simulink model "HW4"  (R2023b)
settings: Solver=FixedStepAuto  StartTime=0.0  StopTime=100  FixedStep=0.5  RelTol=1e-3
settings Model: Creator=ArshiaGosh  LastModifiedBy=ArshiaGosh

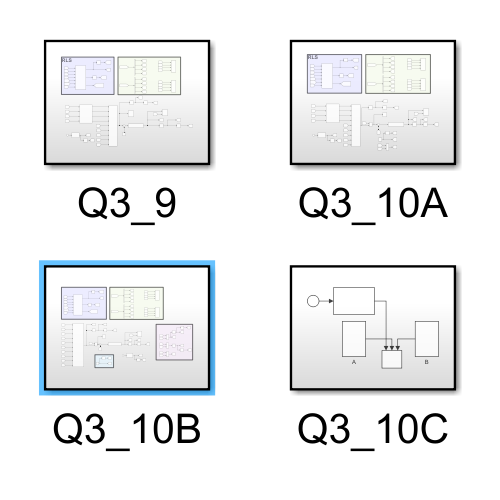
[thumbnail: Simulink's stored preview of the top-level diagram]
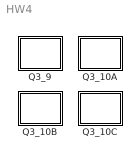
== system HW4 ==
  Q3_10A : Subsystem
  Q3_10B : Subsystem
  Q3_10C : Subsystem
  Q3_9 : Subsystem

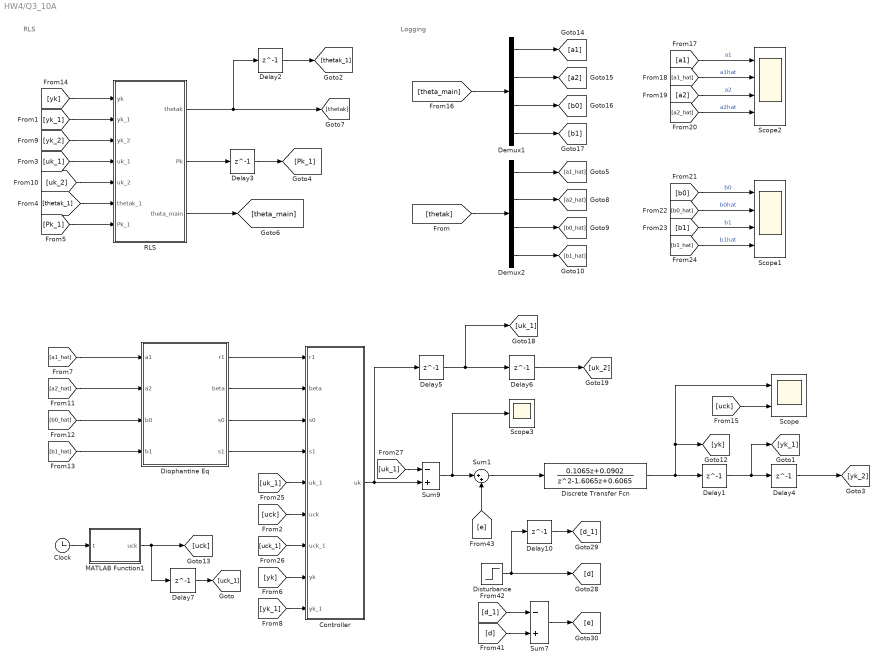
== system HW4/Q3_10A ==
  note: RLS
  note: Logging
  Clock : Clock
  Controller : MATLAB Function  TreatAsAtomicUnit=on
  Delay{1,4..7,10} (6 alike) : Delay  DelayLength=1
  Delay2 : Delay  DelayLength=1  InitialCondition=[0;0;0.01;0.2]
  Delay3 : Delay  DelayLength=1  InitialCondition=[100 0 0 0;0 100 0 0;0 0 1 0;0 0 0 1]
  Demux1 : Demux
  Demux2 : Demux
  Diophantine Eq : MATLAB Function  TreatAsAtomicUnit=on
  Discrete Transfer Fcn : DiscreteTransferFcn  Numerator=[0.1065 0.0902]  Denominator=[1 -1.6065 0.6065]
  Disturbance : Step  Time=40  After=0.5
  MATLAB Function1 : MATLAB Function  TreatAsAtomicUnit=on
  RLS : MATLAB Function  TreatAsAtomicUnit=on
  Scope : Scope  NumInputPorts=2
  Scope1 : Scope  NumInputPorts=4
  Scope2 : Scope  NumInputPorts=4
  Scope3 : Scope
  Sum1 : Sum  Inputs=|++
  Sum7 : Sum  Inputs=-+
  Sum9 : Sum  Inputs=-+
  wires:
  Sum1/1 -> Discrete Transfer Fcn/1
  [uck_1] -> Controller/7(uck_1)
  Delay7/1 -> [uck_1]
  Demux2/1 -> [a1_hat]
  Demux2/2 -> [a2_hat]
  Demux2/4 -> [b1_hat]
  Demux2/3 -> [b0_hat]
  [thetak] -> Demux2/1
  Delay6/1 -> [uk_2]
  [uk_1] -> Controller/5(uk_1)
  Delay5/1 -> Delay6/1, [uk_1]
  [yk] -> RLS/1(yk)
  [yk_1] -> Controller/9(yk_1)
  [yk] -> Controller/8(yk)
  [uck] -> Controller/6(uck)
  Clock/1 -> MATLAB Function1/1(t)
  MATLAB Function1/1(uck) -> Delay7/1, [uck]
  Diophantine Eq/4(s1) -> Controller/4(s1)
  Diophantine Eq/1(r1) -> Controller/1(r1)
  Diophantine Eq/2(beta) -> Controller/2(beta)
  Diophantine Eq/3(s0) -> Controller/3(s0)
  [b1] -> Scope1/3  "b1"
  [b1_hat] -> Scope1/4  "b1hat"
  [b0_hat] -> Scope1/2  "b0hat"
  [b0] -> Scope1/1  "b0"
  [a2_hat] -> Scope2/4  "a2hat"
  [a2] -> Scope2/3  "a2"
  [a1_hat] -> Scope2/2  "a1hat"
  [a1] -> Scope2/1  "a1"
  Demux1/1 -> [a1]
  [theta_main] -> Demux1/1
  [uk_1] -> RLS/4(uk_1)
  Demux1/4 -> [b1]
  Demux1/3 -> [b0]
  RLS/2(Pk) -> Delay3/1
  [a2_hat] -> Diophantine Eq/2(a2)
  [thetak_1] -> RLS/6(thetak_1)
  Demux1/2 -> [a2]
  Delay1/1 -> Delay4/1, [yk_1]
  [uk_2] -> RLS/5(uk_2)
  [uck] -> Scope/2
  Delay3/1 -> [Pk_1]
  RLS/1(thetak) -> [thetak], Delay2/1
  [yk_1] -> RLS/2(yk_1)
  Delay2/1 -> [thetak_1]
  [Pk_1] -> RLS/7(Pk_1)
  RLS/3(theta_main) -> [theta_main]
  [b1_hat] -> Diophantine Eq/4(b1)
  [a1_hat] -> Diophantine Eq/1(a1)
  [b0_hat] -> Diophantine Eq/3(b0)
  Delay4/1 -> [yk_2]
  Discrete Transfer Fcn/1 -> Delay1/1, [yk], Scope/1
  [yk_2] -> RLS/3(yk_2)
  Disturbance/1 -> [d], Delay10/1
  Delay10/1 -> [d_1]
  Sum7/1 -> [e]
  [d_1] -> Sum7/1
  [d] -> Sum7/2
  [e] -> Sum1/2
  Controller/1(uk) -> Delay5/1, Sum9/2
  [uk_1] -> Sum9/1
  Sum9/1 -> Scope3/1, Sum1/1

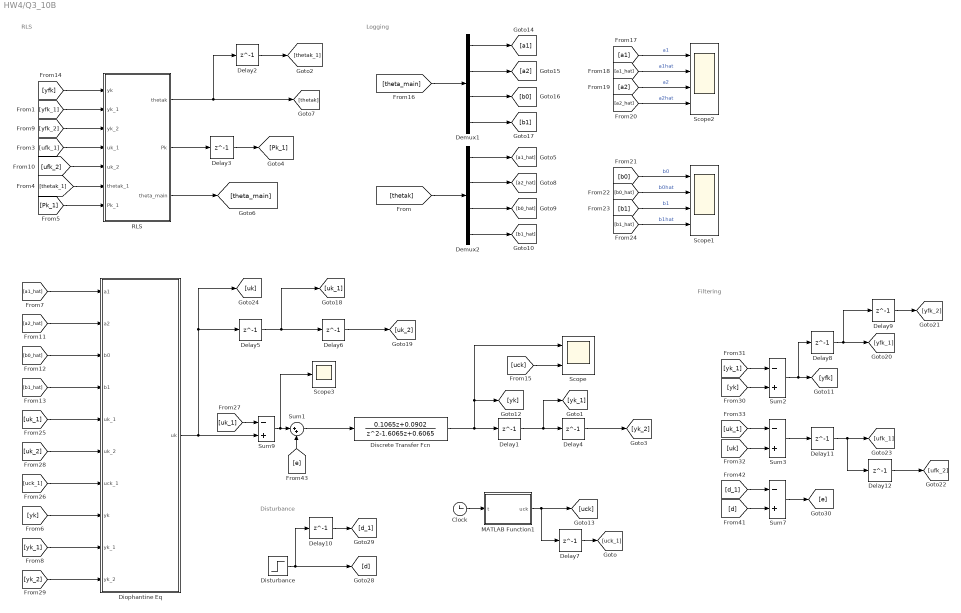
== system HW4/Q3_10B ==
  note: Filtering
  note: Disturbance
  note: Logging
  note: RLS
  Clock : Clock
  Delay{1,4..12} (10 alike) : Delay  DelayLength=1
  Delay2 : Delay  DelayLength=1  InitialCondition=[0;0;0.01;0.2]
  Delay3 : Delay  DelayLength=1  InitialCondition=[100 0 0 0;0 100 0 0;0 0 1 0;0 0 0 1]
  Demux1 : Demux
  Demux2 : Demux
  Diophantine Eq : MATLAB Function  TreatAsAtomicUnit=on
  Discrete Transfer Fcn : DiscreteTransferFcn  Numerator=[0.1065 0.0902]  Denominator=[1 -1.6065 0.6065]
  Disturbance : Step  Time=40  After=0.5
  MATLAB Function1 : MATLAB Function  TreatAsAtomicUnit=on
  RLS : MATLAB Function  TreatAsAtomicUnit=on
  Scope : Scope  NumInputPorts=2
  Scope1 : Scope  NumInputPorts=4
  Scope2 : Scope  NumInputPorts=4
  Scope3 : Scope
  Sum1 : Sum  Inputs=|++
  Sum{2..3,7,9} (4 alike) : Sum  Inputs=-+
  wires:
  Sum9/1 -> Scope3/1, Sum1/1
  [uk_1] -> Sum9/1
  Diophantine Eq/1(uk) -> Sum9/2, [uk], Delay5/1
  [e] -> Sum1/2
  [d] -> Sum7/2
  [d_1] -> Sum7/1
  Sum7/1 -> [e]
  Delay10/1 -> [d_1]
  Disturbance/1 -> Delay10/1, [d]
  [yfk_2] -> RLS/3(yk_2)
  Discrete Transfer Fcn/1 -> Scope/1, [yk], Delay1/1
  Delay4/1 -> [yk_2]
  [b0_hat] -> Diophantine Eq/3(b0)
  [a1_hat] -> Diophantine Eq/1(a1)
  [b1_hat] -> Diophantine Eq/4(b1)
  RLS/3(theta_main) -> [theta_main]
  [Pk_1] -> RLS/7(Pk_1)
  Delay2/1 -> [thetak_1]
  [yfk_1] -> RLS/2(yk_1)
  RLS/1(thetak) -> Delay2/1, [thetak]
  Delay3/1 -> [Pk_1]
  [uck] -> Scope/2
  [ufk_2] -> RLS/5(uk_2)
  Delay1/1 -> [yk_1], Delay4/1
  Demux1/2 -> [a2]
  [thetak_1] -> RLS/6(thetak_1)
  [a2_hat] -> Diophantine Eq/2(a2)
  RLS/2(Pk) -> Delay3/1
  Demux1/3 -> [b0]
  Demux1/4 -> [b1]
  [ufk_1] -> RLS/4(uk_1)
  [theta_main] -> Demux1/1
  Demux1/1 -> [a1]
  [a1] -> Scope2/1  "a1"
  [a1_hat] -> Scope2/2  "a1hat"
  [a2] -> Scope2/3  "a2"
  [a2_hat] -> Scope2/4  "a2hat"
  [b0] -> Scope1/1  "b0"
  [b0_hat] -> Scope1/2  "b0hat"
  [b1_hat] -> Scope1/4  "b1hat"
  [b1] -> Scope1/3  "b1"
  MATLAB Function1/1(uck) -> [uck], Delay7/1
  Clock/1 -> MATLAB Function1/1(t)
  [yk] -> Diophantine Eq/8(yk)
  [yk_1] -> Diophantine Eq/9(yk_1)
  [yfk] -> RLS/1(yk)
  Delay5/1 -> [uk_1], Delay6/1
  [uk_1] -> Diophantine Eq/5(uk_1)
  Delay6/1 -> [uk_2]
  [thetak] -> Demux2/1
  Demux2/3 -> [b0_hat]
  Demux2/4 -> [b1_hat]
  Demux2/2 -> [a2_hat]
  Demux2/1 -> [a1_hat]
  Delay7/1 -> [uck_1]
  [uck_1] -> Diophantine Eq/7(uck_1)
  Sum1/1 -> Discrete Transfer Fcn/1
  [uk_2] -> Diophantine Eq/6(uk_2)
  [yk_2] -> Diophantine Eq/10(yk_2)
  [yk_1] -> Sum2/1
  [yk] -> Sum2/2
  Sum2/1 -> Delay8/1, [yfk]
  Delay8/1 -> Delay9/1, [yfk_1]
  Delay9/1 -> [yfk_2]
  Delay11/1 -> Delay12/1, [ufk_1]
  Sum3/1 -> Delay11/1
  [uk] -> Sum3/2
  [uk_1] -> Sum3/1
  Delay12/1 -> [ufk_2]

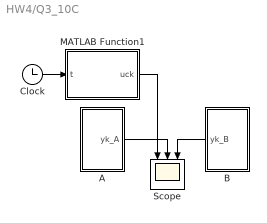
== system HW4/Q3_10C ==
  A : Subsystem
  B : Subsystem
      settings: PortSchema="{\"entries\":[{\"content\":{\"sides\":[{\"content\":{\"connectorIds\":[\"Out1\"]},\"type\":\"ConnectorPlacement.EquallySpacedRectSide\",\"uuid\":\"4f90996b-bf63-4a50-8d94-8952ba228368\"},{\"content\":{\"side\":\"RIGHT\"},\"type\":\"ConnectorPlacement.EquallySpacedRectSide\",\"uuid\":\"625474cf-f28b-4634-93bc-e9f332806dcd\"},{\"content\":{\"side\":\"TOP\"},\"type\":\"ConnectorPlacement.EquallySpacedRectSide\",\"uuid\":\"4c167490-54dc-429f-a938-d7ec9c5d3cf4\"}]},\"type\":\"ConnectorPlacement.EquallySpacedConnector\",\"uuid\":\"62c82442-9d1b-46d0-bbef-764c1c26d001\"}],\"packageUris\":[\"http://schema.mathworks.com/mf0/Connector/R2020b\"],\"version\":\"1.0\"}"
  Clock : Clock
  MATLAB Function1 : MATLAB Function  TreatAsAtomicUnit=on
  Scope : Scope  NumInputPorts=3
  wires:
  A/1(yk_A) -> Scope/2
  B/1(yk_B) -> Scope/3
  MATLAB Function1/1(uck) -> Scope/1
  Clock/1 -> MATLAB Function1/1(t)

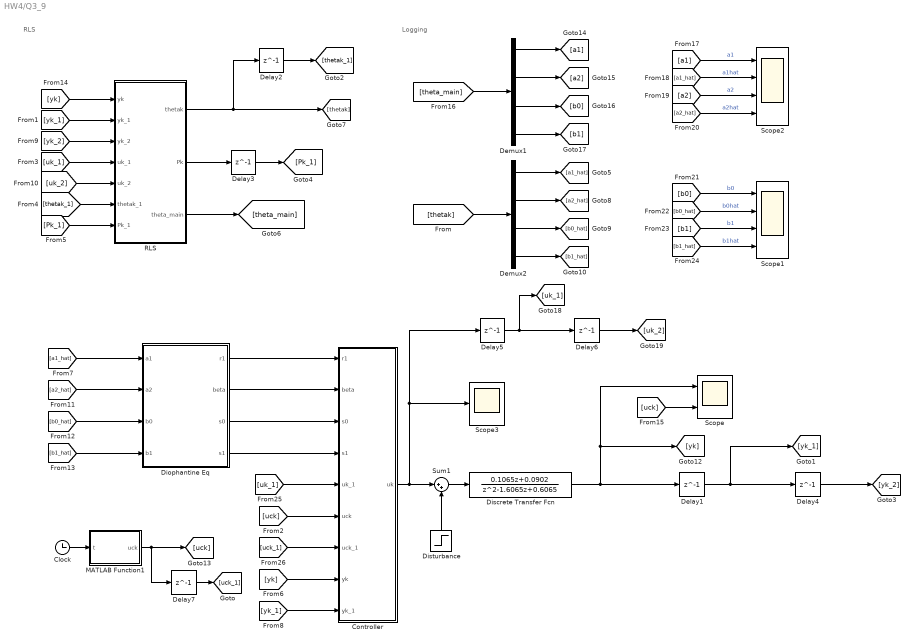
== system HW4/Q3_9 ==
  note: Logging
  note: RLS
  Clock : Clock
  Controller : MATLAB Function  TreatAsAtomicUnit=on
  Delay{1,4..7} (5 alike) : Delay  DelayLength=1
  Delay2 : Delay  DelayLength=1  InitialCondition=[0;0;0.01;0.2]
  Delay3 : Delay  DelayLength=1  InitialCondition=[100 0 0 0;0 100 0 0;0 0 1 0;0 0 0 1]
  Demux1 : Demux
  Demux2 : Demux
  Diophantine Eq : MATLAB Function  TreatAsAtomicUnit=on
  Discrete Transfer Fcn : DiscreteTransferFcn  Numerator=[0.1065 0.0902]  Denominator=[1 -1.6065 0.6065]
  Disturbance : Step  Time=40  After=+0.5
  MATLAB Function1 : MATLAB Function  TreatAsAtomicUnit=on
  RLS : MATLAB Function  TreatAsAtomicUnit=on
  Scope : Scope  NumInputPorts=2
  Scope1 : Scope  NumInputPorts=4
  Scope2 : Scope  NumInputPorts=4
  Scope3 : Scope
  Sum1 : Sum  Inputs=|++
  wires:
  [yk_2] -> RLS/3(yk_2)
  Discrete Transfer Fcn/1 -> Scope/1, [yk], Delay1/1
  Delay4/1 -> [yk_2]
  [b0_hat] -> Diophantine Eq/3(b0)
  [a1_hat] -> Diophantine Eq/1(a1)
  [b1_hat] -> Diophantine Eq/4(b1)
  RLS/3(theta_main) -> [theta_main]
  [Pk_1] -> RLS/7(Pk_1)
  Delay2/1 -> [thetak_1]
  [yk_1] -> RLS/2(yk_1)
  RLS/1(thetak) -> Delay2/1, [thetak]
  Delay3/1 -> [Pk_1]
  [uck] -> Scope/2
  [uk_2] -> RLS/5(uk_2)
  Delay1/1 -> Delay4/1, [yk_1]
  Demux1/2 -> [a2]
  [thetak_1] -> RLS/6(thetak_1)
  [a2_hat] -> Diophantine Eq/2(a2)
  RLS/2(Pk) -> Delay3/1
  Demux1/3 -> [b0]
  Demux1/4 -> [b1]
  [uk_1] -> RLS/4(uk_1)
  [theta_main] -> Demux1/1
  Demux1/1 -> [a1]
  [a1] -> Scope2/1  "a1"
  [a1_hat] -> Scope2/2  "a1hat"
  [a2] -> Scope2/3  "a2"
  [a2_hat] -> Scope2/4  "a2hat"
  [b0] -> Scope1/1  "b0"
  [b0_hat] -> Scope1/2  "b0hat"
  [b1_hat] -> Scope1/4  "b1hat"
  [b1] -> Scope1/3  "b1"
  Diophantine Eq/3(s0) -> Controller/3(s0)
  Diophantine Eq/2(beta) -> Controller/2(beta)
  Diophantine Eq/1(r1) -> Controller/1(r1)
  Diophantine Eq/4(s1) -> Controller/4(s1)
  MATLAB Function1/1(uck) -> [uck], Delay7/1
  Clock/1 -> MATLAB Function1/1(t)
  [uck] -> Controller/6(uck)
  [yk] -> Controller/8(yk)
  [yk_1] -> Controller/9(yk_1)
  [yk] -> RLS/1(yk)
  Delay5/1 -> Delay6/1, [uk_1]
  [uk_1] -> Controller/5(uk_1)
  Delay6/1 -> [uk_2]
  Controller/1(uk) -> Delay5/1, Scope3/1, Sum1/1
  [thetak] -> Demux2/1
  Demux2/3 -> [b0_hat]
  Demux2/4 -> [b1_hat]
  Demux2/2 -> [a2_hat]
  Demux2/1 -> [a1_hat]
  Delay7/1 -> [uck_1]
  [uck_1] -> Controller/7(uck_1)
  Sum1/1 -> Discrete Transfer Fcn/1
  Disturbance/1 -> Sum1/2

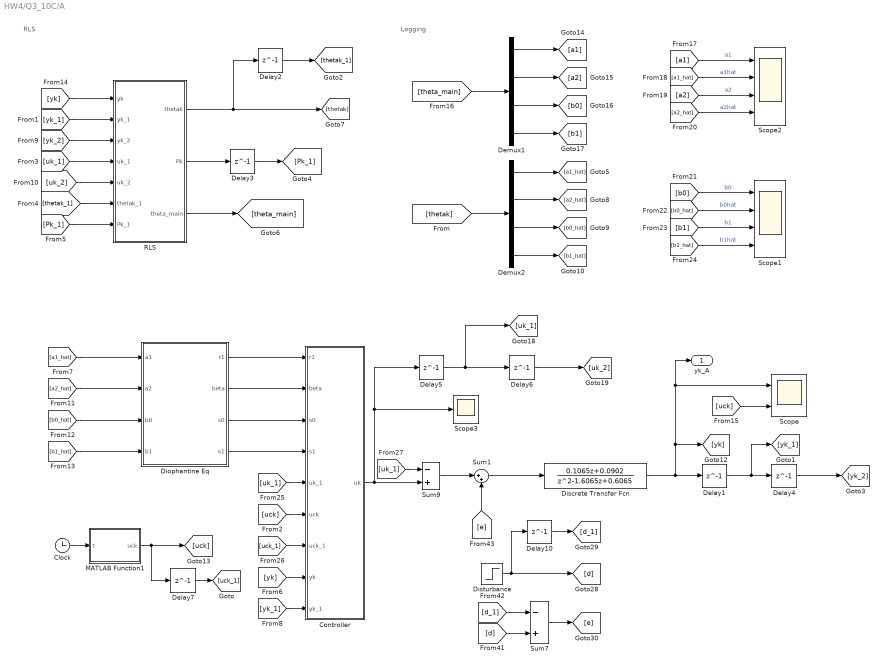
== system HW4/Q3_10C/A ==
  note: Logging
  note: RLS
  Clock : Clock
  Controller : MATLAB Function  TreatAsAtomicUnit=on
  Delay{1,4..7,10} (6 alike) : Delay  DelayLength=1
  Delay2 : Delay  DelayLength=1  InitialCondition=[0;0;0.01;0.2]
  Delay3 : Delay  DelayLength=1  InitialCondition=[100 0 0 0;0 100 0 0;0 0 1 0;0 0 0 1]
  Demux1 : Demux
  Demux2 : Demux
  Diophantine Eq : MATLAB Function  TreatAsAtomicUnit=on
  Discrete Transfer Fcn : DiscreteTransferFcn  Numerator=[0.1065 0.0902]  Denominator=[1 -1.6065 0.6065]
  Disturbance : Step  Time=40  After=0.5
  MATLAB Function1 : MATLAB Function  TreatAsAtomicUnit=on
  RLS : MATLAB Function  TreatAsAtomicUnit=on
  Scope : Scope  NumInputPorts=2
  Scope1 : Scope  NumInputPorts=4
  Scope2 : Scope  NumInputPorts=4
  Scope3 : Scope
  Sum1 : Sum  Inputs=|++
  Sum7 : Sum  Inputs=-+
  Sum9 : Sum  Inputs=-+
  yk_A : Outport
  wires:
  [uck] -> Scope/2
  [b0_hat] -> Scope1/2  "b0hat"
  Delay4/1 -> [yk_2]
  Delay2/1 -> [thetak_1]
  [d_1] -> Sum7/1
  Delay7/1 -> [uck_1]
  [a1_hat] -> Scope2/2  "a1hat"
  [yk_2] -> RLS/3(yk_2)
  [Pk_1] -> RLS/7(Pk_1)
  Delay3/1 -> [Pk_1]
  [thetak_1] -> RLS/6(thetak_1)
  [a2_hat] -> Diophantine Eq/2(a2)
  [d] -> Sum7/2
  Diophantine Eq/3(s0) -> Controller/3(s0)
  Sum7/1 -> [e]
  [uck] -> Controller/6(uck)
  Demux1/4 -> [b1]
  [b1] -> Scope1/3  "b1"
  RLS/1(thetak) -> [thetak], Delay2/1
  [a2_hat] -> Scope2/4  "a2hat"
  [uk_2] -> RLS/5(uk_2)
  Disturbance/1 -> [d], Delay10/1
  [b0_hat] -> Diophantine Eq/3(b0)
  [thetak] -> Demux2/1
  RLS/2(Pk) -> Delay3/1
  Controller/1(uk) -> Delay5/1, Scope3/1, Sum9/2
  [yk] -> Controller/8(yk)
  Diophantine Eq/1(r1) -> Controller/1(r1)
  Discrete Transfer Fcn/1 -> Delay1/1, [yk], yk_A/1, Scope/1
  Diophantine Eq/4(s1) -> Controller/4(s1)
  MATLAB Function1/1(uck) -> Delay7/1, [uck]
  [yk_1] -> Controller/9(yk_1)
  [a2] -> Scope2/3  "a2"
  Delay1/1 -> Delay4/1, [yk_1]
  Demux1/1 -> [a1]
  [yk_1] -> RLS/2(yk_1)
  Demux1/2 -> [a2]
  [uk_1] -> RLS/4(uk_1)
  Sum1/1 -> Discrete Transfer Fcn/1
  Demux2/2 -> [a2_hat]
  [uk_1] -> Sum9/1
  Diophantine Eq/2(beta) -> Controller/2(beta)
  [b1_hat] -> Scope1/4  "b1hat"
  [a1] -> Scope2/1  "a1"
  [a1_hat] -> Diophantine Eq/1(a1)
  [uk_1] -> Controller/5(uk_1)
  [uck_1] -> Controller/7(uck_1)
  Demux2/1 -> [a1_hat]
  RLS/3(theta_main) -> [theta_main]
  Demux2/3 -> [b0_hat]
  [theta_main] -> Demux1/1
  Delay10/1 -> [d_1]
  [yk] -> RLS/1(yk)
  Demux2/4 -> [b1_hat]
  [b1_hat] -> Diophantine Eq/4(b1)
  Delay6/1 -> [uk_2]
  [e] -> Sum1/2
  Delay5/1 -> Delay6/1, [uk_1]
  Sum9/1 -> Sum1/1
  [b0] -> Scope1/1  "b0"
  Demux1/3 -> [b0]
  Clock/1 -> MATLAB Function1/1(t)

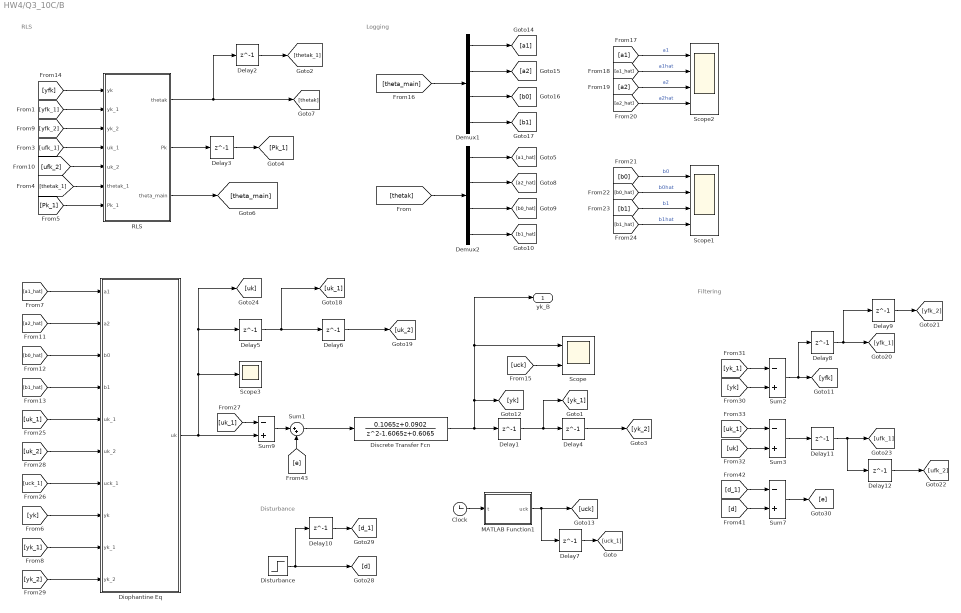
== system HW4/Q3_10C/B ==
  note: Filtering
  note: Disturbance
  note: Logging
  note: RLS
  Clock : Clock
  Delay{1,4..12} (10 alike) : Delay  DelayLength=1
  Delay2 : Delay  DelayLength=1  InitialCondition=[0;0;0.01;0.2]
  Delay3 : Delay  DelayLength=1  InitialCondition=[100 0 0 0;0 100 0 0;0 0 1 0;0 0 0 1]
  Demux1 : Demux
  Demux2 : Demux
  Diophantine Eq : MATLAB Function  TreatAsAtomicUnit=on
  Discrete Transfer Fcn : DiscreteTransferFcn  Numerator=[0.1065 0.0902]  Denominator=[1 -1.6065 0.6065]
  Disturbance : Step  Time=40  After=0.5
  MATLAB Function1 : MATLAB Function  TreatAsAtomicUnit=on
  RLS : MATLAB Function  TreatAsAtomicUnit=on
  Scope : Scope  NumInputPorts=2
  Scope1 : Scope  NumInputPorts=4
  Scope2 : Scope  NumInputPorts=4
  Scope3 : Scope
  Sum1 : Sum  Inputs=|++
  Sum{2..3,7,9} (4 alike) : Sum  Inputs=-+
  yk_B : Outport
  wires:
  Sum9/1 -> Sum1/1
  [uk_1] -> Sum9/1
  Diophantine Eq/1(uk) -> Sum9/2, [uk], Delay5/1, Scope3/1
  [e] -> Sum1/2
  [d] -> Sum7/2
  [d_1] -> Sum7/1
  Sum7/1 -> [e]
  Delay10/1 -> [d_1]
  Disturbance/1 -> Delay10/1, [d]
  [yfk_2] -> RLS/3(yk_2)
  Discrete Transfer Fcn/1 -> Scope/1, yk_B/1, [yk], Delay1/1
  Delay4/1 -> [yk_2]
  [b0_hat] -> Diophantine Eq/3(b0)
  [a1_hat] -> Diophantine Eq/1(a1)
  [b1_hat] -> Diophantine Eq/4(b1)
  RLS/3(theta_main) -> [theta_main]
  [Pk_1] -> RLS/7(Pk_1)
  Delay2/1 -> [thetak_1]
  [yfk_1] -> RLS/2(yk_1)
  RLS/1(thetak) -> Delay2/1, [thetak]
  Delay3/1 -> [Pk_1]
  [uck] -> Scope/2
  [ufk_2] -> RLS/5(uk_2)
  Delay1/1 -> [yk_1], Delay4/1
  Demux1/2 -> [a2]
  [thetak_1] -> RLS/6(thetak_1)
  [a2_hat] -> Diophantine Eq/2(a2)
  RLS/2(Pk) -> Delay3/1
  Demux1/3 -> [b0]
  Demux1/4 -> [b1]
  [ufk_1] -> RLS/4(uk_1)
  [theta_main] -> Demux1/1
  Demux1/1 -> [a1]
  [a1] -> Scope2/1  "a1"
  [a1_hat] -> Scope2/2  "a1hat"
  [a2] -> Scope2/3  "a2"
  [a2_hat] -> Scope2/4  "a2hat"
  [b0] -> Scope1/1  "b0"
  [b0_hat] -> Scope1/2  "b0hat"
  [b1_hat] -> Scope1/4  "b1hat"
  [b1] -> Scope1/3  "b1"
  MATLAB Function1/1(uck) -> [uck], Delay7/1
  Clock/1 -> MATLAB Function1/1(t)
  [yk] -> Diophantine Eq/8(yk)
  [yk_1] -> Diophantine Eq/9(yk_1)
  [yfk] -> RLS/1(yk)
  Delay5/1 -> [uk_1], Delay6/1
  [uk_1] -> Diophantine Eq/5(uk_1)
  Delay6/1 -> [uk_2]
  [thetak] -> Demux2/1
  Demux2/3 -> [b0_hat]
  Demux2/4 -> [b1_hat]
  Demux2/2 -> [a2_hat]
  Demux2/1 -> [a1_hat]
  Delay7/1 -> [uck_1]
  [uck_1] -> Diophantine Eq/7(uck_1)
  Sum1/1 -> Discrete Transfer Fcn/1
  [uk_2] -> Diophantine Eq/6(uk_2)
  [yk_2] -> Diophantine Eq/10(yk_2)
  [yk_1] -> Sum2/1
  [yk] -> Sum2/2
  Sum2/1 -> Delay8/1, [yfk]
  Delay8/1 -> Delay9/1, [yfk_1]
  Delay9/1 -> [yfk_2]
  Delay11/1 -> Delay12/1, [ufk_1]
  Sum3/1 -> Delay11/1
  [uk] -> Sum3/2
  [uk_1] -> Sum3/1
  Delay12/1 -> [ufk_2]

== matlab function HW4/Q3_9/MATLAB Function1 ==
  data: t input; uck output
function uck = fcn(t)
if t>=0 && t<25
    uck=1;
elseif t>=25 && t<50
    uck=-1;
elseif t>=50 && t<75
    uck=1;
else
    uck=-1;
end

== matlab function HW4/Q3_9/RLS ==
  data: yk input; yk_1 input; yk_2 input; uk_1 input; uk_2 input; thetak_1 input; Pk_1 input; thetak output; Pk output; theta_main output
function [thetak,Pk,theta_main] = fcn(yk, yk_1,yk_2,uk_1,uk_2,thetak_1,Pk_1)
a1 = -1.6065;
a2 = 0.6065;
b0 = 0.1065;
b1 = 0.0902;
theta_main=[a1;a2;b0;b1];

%estimate
lambda = 0.98;
phi = [-yk_1; -yk_2; uk_1; uk_2];
Kk = (Pk_1 * phi) / (lambda + phi' * Pk_1 * phi);
Pk = (1/lambda) * (Pk_1 - Kk * phi' * Pk_1);
thetak = thetak_1 + Kk * (yk - phi' * thetak_1);

== matlab function HW4/Q3_10C/A/Controller ==
  data: r1 input; uk output; beta input; s0 input; s1 input; uk_1 input; uck input; uck_1 input; yk input; yk_1 input
function uk = fcn(r1,beta, s0,s1,uk_1, uck, uck_1,yk,yk_1)
a0=0;
uk= - uk_1*r1+beta*uck+beta*a0*uck_1-s0*yk-s1*yk_1;

== matlab function HW4/Q3_10B/Diophantine Eq ==
  data: a1 input; a2 input; b0 input; b1 input; uk output; uk_1 input; uk_2 input; uck_1 input; yk input; yk_1 input; yk_2 input
function uk = fcn(a1,a2,b0,b1,uk_1,uk_2,uck_1, yk, yk_1,yk_2)
am1=-1.3205;
am2=0.4966;
beta=(1+am1+am2)/(b0+b1);
a0=0;
r1=(a0*am2*b0^2+(a2-am2-a0*am1)*b0*b1+(a0+am1-a1)*b1^2)/(b1^2-a1*b0*b1+a2*b0^2);
s0=(b1*(a0*am1-a2-am1*a1+a1^2+am2-a1*a0)+b0*(am1*a2-a1*a2-a0*am2+a0*a2))/(b1^2-a1*b0*b1+a2*b0^2);
s1=(b1*(a1*a2-am1*a2+a0*am2-a0*a2)+b0*(a2*am2-a2^2-a0*am2*a1-a0*a2*am1))/(b1^2-a1*b0*b1+a2*b0^2);
t0=beta;
y0 = (- (1+r1))/(b0+b1);
uk=-r1*uk_1- y0*b0*uk_1 - y0*b1*uk_2 + t0*uck_1 - (s0*yk + s1*yk_1 - y0*yk-a1*y0*yk_1 - y0*a2*yk_2);
end

== matlab function HW4/Q3_10B/MATLAB Function1 ==
  data: t input; uck output
function uck = fcn(t)
if t>=0 && t<25
    uck=1;
elseif t>=25 && t<50
    uck=-1;
elseif t>=50 && t<75
    uck=1;
else
    uck=-1;
end

== matlab function HW4/Q3_10B/RLS ==
  data: yk input; yk_1 input; yk_2 input; uk_1 input; uk_2 input; thetak_1 input; Pk_1 input; thetak output; Pk output; theta_main output
function [thetak,Pk,theta_main] = fcn(yk, yk_1,yk_2,uk_1,uk_2,thetak_1,Pk_1)
a1 = -1.6065;
a2 = 0.6065;
b0 = 0.1065;
b1 = 0.0902;
theta_main=[a1;a2;b0;b1];

%estimate
lambda = 0.98;
phi = [-yk_1; -yk_2; uk_1; uk_2];
Kk = (Pk_1 * phi) / (lambda + phi' * Pk_1 * phi);
Pk = (1/lambda) * (Pk_1 - Kk * phi' * Pk_1);
thetak = thetak_1 + Kk * (yk - phi' * thetak_1);

== matlab function HW4/Q3_10C/A/Diophantine Eq ==
  data: r1 output; beta output; s0 output; s1 output; a1 input; a2 input; b0 input; b1 input
function [r1,beta,s0,s1]   = fcn(a1,a2,b0,b1)
am1=-1.3205;
am2=0.4966;
bm0=0.1761;
beta=(1+am1+am2)/(b0+b1);
bm0=beta*b0;
a0=0;
r1=(a0*am2*b0^2+(a2-am2-a0*am1)*b0*b1+(a0+am1-a1)*b1^2)/(b1^2-a1*b0*b1+a2*b0^2);
s0=(b1*(a0*am1-a2-am1*a1+a1^2+am2-a1*a0)+b0*(am1*a2-a1*a2-a0*am2+a0*a2))/(b1^2-a1*b0*b1+a2*b0^2);
s1=(b1*(a1*a2-am1*a2+a0*am2-a0*a2)+b0*(a2*am2-a2^2-a0*am2*a1-a0*a2*am1))/(b1^2-a1*b0*b1+a2*b0^2);

== matlab function HW4/Q3_10C/A/MATLAB Function1 ==
  data: t input; uck output
function uck = fcn(t)
if t>=0 && t<25
    uck=1;
elseif t>=25 && t<50
    uck=-1;
elseif t>=50 && t<75
    uck=1;
else
    uck=-1;
end

== matlab function HW4/Q3_10C/A/RLS ==
  data: yk input; yk_1 input; yk_2 input; uk_1 input; uk_2 input; thetak_1 input; Pk_1 input; thetak output; Pk output; theta_main output
function [thetak,Pk,theta_main] = fcn(yk, yk_1,yk_2,uk_1,uk_2,thetak_1,Pk_1)
a1 = -1.6065;
a2 = 0.6065;
b0 = 0.1065;
b1 = 0.0902;
theta_main=[a1;a2;b0;b1];

%estimate
lambda = 0.98;
phi = [-yk_1; -yk_2; uk_1; uk_2];
Kk = (Pk_1 * phi) / (lambda + phi' * Pk_1 * phi);
Pk = (1/lambda) * (Pk_1 - Kk * phi' * Pk_1);
thetak = thetak_1 + Kk * (yk - phi' * thetak_1);

== matlab function HW4/Q3_10C/B/Diophantine Eq ==
  data: a1 input; a2 input; b0 input; b1 input; uk output; uk_1 input; uk_2 input; uck_1 input; yk input; yk_1 input; yk_2 input
function uk = fcn(a1,a2,b0,b1,uk_1,uk_2,uck_1, yk, yk_1,yk_2)
am1=-1.3205;
am2=0.4966;
beta=(1+am1+am2)/(b0+b1);
a0=0;
r1=(a0*am2*b0^2+(a2-am2-a0*am1)*b0*b1+(a0+am1-a1)*b1^2)/(b1^2-a1*b0*b1+a2*b0^2);
s0=(b1*(a0*am1-a2-am1*a1+a1^2+am2-a1*a0)+b0*(am1*a2-a1*a2-a0*am2+a0*a2))/(b1^2-a1*b0*b1+a2*b0^2);
s1=(b1*(a1*a2-am1*a2+a0*am2-a0*a2)+b0*(a2*am2-a2^2-a0*am2*a1-a0*a2*am1))/(b1^2-a1*b0*b1+a2*b0^2);
t0=beta;
y0 = (- (1+r1))/(b0+b1);
uk=-r1*uk_1- y0*b0*uk_1 - y0*b1*uk_2 + t0*uck_1 - (s0*yk + s1*yk_1 - y0*yk-a1*y0*yk_1 - y0*a2*yk_2);
end

== matlab function HW4/Q3_10C/B/MATLAB Function1 ==
  data: t input; uck output
function uck = fcn(t)
if t>=0 && t<25
    uck=1;
elseif t>=25 && t<50
    uck=-1;
elseif t>=50 && t<75
    uck=1;
else
    uck=-1;
end

== matlab function HW4/Q3_10C/B/RLS ==
  data: yk input; yk_1 input; yk_2 input; uk_1 input; uk_2 input; thetak_1 input; Pk_1 input; thetak output; Pk output; theta_main output
function [thetak,Pk,theta_main] = fcn(yk, yk_1,yk_2,uk_1,uk_2,thetak_1,Pk_1)
a1 = -1.6065;
a2 = 0.6065;
b0 = 0.1065;
b1 = 0.0902;
theta_main=[a1;a2;b0;b1];

%estimate
lambda = 0.98;
phi = [-yk_1; -yk_2; uk_1; uk_2];
Kk = (Pk_1 * phi) / (lambda + phi' * Pk_1 * phi);
Pk = (1/lambda) * (Pk_1 - Kk * phi' * Pk_1);
thetak = thetak_1 + Kk * (yk - phi' * thetak_1);

== matlab function HW4/Q3_10C/MATLAB Function1 ==
  data: t input; uck output
function uck = fcn(t)
if t>=0 && t<25
    uck=1;
elseif t>=25 && t<50
    uck=-1;
elseif t>=50 && t<75
    uck=1;
else
    uck=-1;
end

== matlab function HW4/Q3_10A/Controller ==
  data: r1 input; uk output; beta input; s0 input; s1 input; uk_1 input; uck input; uck_1 input; yk input; yk_1 input
function uk = fcn(r1,beta, s0,s1,uk_1, uck, uck_1,yk,yk_1)
a0=0;
uk= - uk_1*r1+beta*uck+beta*a0*uck_1-s0*yk-s1*yk_1;

== matlab function HW4/Q3_10A/Diophantine Eq ==
  data: r1 output; beta output; s0 output; s1 output; a1 input; a2 input; b0 input; b1 input
function [r1,beta,s0,s1]   = fcn(a1,a2,b0,b1)
am1=-1.3205;
am2=0.4966;
bm0=0.1761;
beta=(1+am1+am2)/(b0+b1);
bm0=beta*b0;
a0=0;
r1=(a0*am2*b0^2+(a2-am2-a0*am1)*b0*b1+(a0+am1-a1)*b1^2)/(b1^2-a1*b0*b1+a2*b0^2);
s0=(b1*(a0*am1-a2-am1*a1+a1^2+am2-a1*a0)+b0*(am1*a2-a1*a2-a0*am2+a0*a2))/(b1^2-a1*b0*b1+a2*b0^2);
s1=(b1*(a1*a2-am1*a2+a0*am2-a0*a2)+b0*(a2*am2-a2^2-a0*am2*a1-a0*a2*am1))/(b1^2-a1*b0*b1+a2*b0^2);

== matlab function HW4/Q3_9/Controller ==
  data: r1 input; uk output; beta input; s0 input; s1 input; uk_1 input; uck input; uck_1 input; yk input; yk_1 input
function uk = fcn(r1,beta, s0,s1,uk_1, uck, uck_1,yk,yk_1)
a0=0;
uk= - uk_1*r1+beta*uck+beta*a0*uck_1-s0*yk-s1*yk_1;

== matlab function HW4/Q3_9/Diophantine Eq ==
  data: r1 output; beta output; s0 output; s1 output; a1 input; a2 input; b0 input; b1 input
function [r1,beta,s0,s1]   = fcn(a1,a2,b0,b1)
am1=-1.3205;
am2=0.4966;
bm0=0.1761;
beta=(1+am1+am2)/(b0+b1);
bm0=beta*b0;
a0=0;
r1=(a0*am2*b0^2+(a2-am2-a0*am1)*b0*b1+(a0+am1-a1)*b1^2)/(b1^2-a1*b0*b1+a2*b0^2);
s0=(b1*(a0*am1-a2-am1*a1+a1^2+am2-a1*a0)+b0*(am1*a2-a1*a2-a0*am2+a0*a2))/(b1^2-a1*b0*b1+a2*b0^2);
s1=(b1*(a1*a2-am1*a2+a0*am2-a0*a2)+b0*(a2*am2-a2^2-a0*am2*a1-a0*a2*am1))/(b1^2-a1*b0*b1+a2*b0^2);

== matlab function HW4/Q3_10A/MATLAB Function1 ==
  data: t input; uck output
function uck = fcn(t)
if t>=0 && t<25
    uck=1;
elseif t>=25 && t<50
    uck=-1;
elseif t>=50 && t<75
    uck=1;
else
    uck=-1;
end

== matlab function HW4/Q3_10A/RLS ==
  data: yk input; yk_1 input; yk_2 input; uk_1 input; uk_2 input; thetak_1 input; Pk_1 input; thetak output; Pk output; theta_main output
function [thetak,Pk,theta_main] = fcn(yk, yk_1,yk_2,uk_1,uk_2,thetak_1,Pk_1)
a1 = -1.6065;
a2 = 0.6065;
b0 = 0.1065;
b1 = 0.0902;
theta_main=[a1;a2;b0;b1];

%estimate
lambda = 0.98;
phi = [-yk_1; -yk_2; uk_1; uk_2];
Kk = (Pk_1 * phi) / (lambda + phi' * Pk_1 * phi);
Pk = (1/lambda) * (Pk_1 - Kk * phi' * Pk_1);
thetak = thetak_1 + Kk * (yk - phi' * thetak_1);
